simulink model "kapizza_pendulum"  (R2023b)
settings: Solver=VariableStepAuto  StartTime=0.0  StopTime=10  MaxStep=0.01  RelTol=1e-3
values from neighbouring files (symbols this model uses):
  Amplitude = 0.1    [kapizza_script.m]
  decrement = 0.3    [kapizza_script.m]
  Frequency = F_0*30    [kapizza_script.m]
  g = 9.8    [kapizza_script.m]
  L = 1    [kapizza_script.m]
  m = 1    [kapizza_script.m]
  start_angle = 120    [kapizza_script.m]
undefined symbols (not defined in the file or in its folder): I
libraries: simulink_extras x2
settings Model: Creator=user  LastModifiedBy=user
settings DataIOCC: ReturnWorkspaceOutputs=off

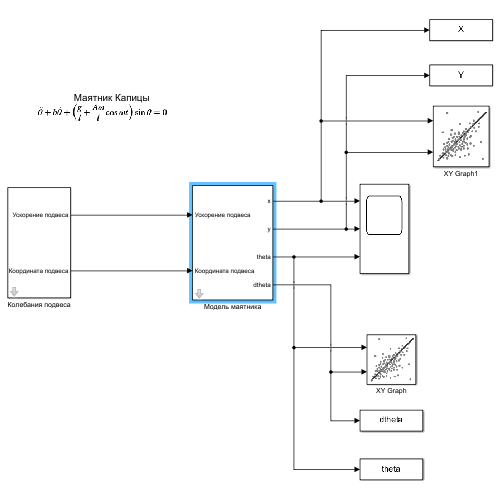
[thumbnail: Simulink's stored preview of the top-level diagram]
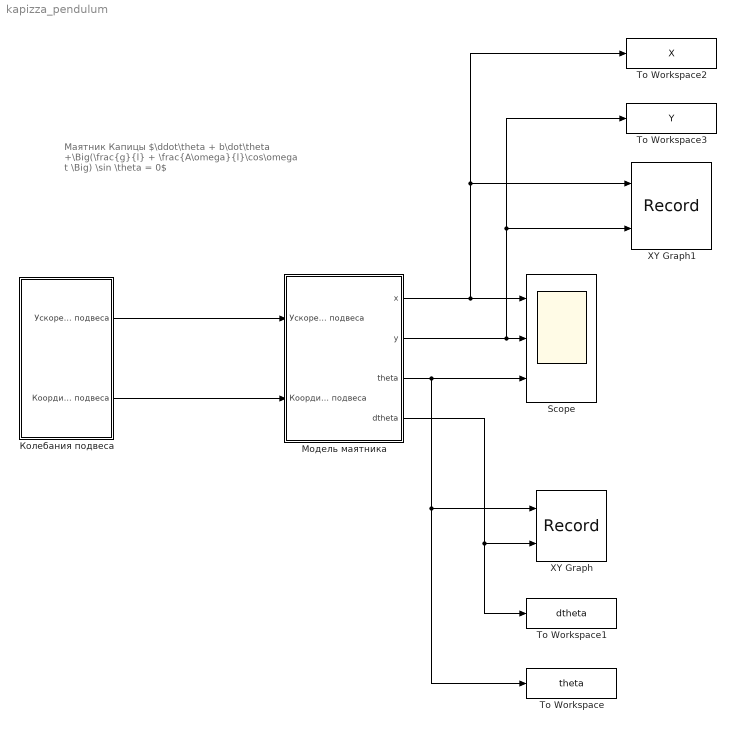
== system kapizza_pendulum ==
  note: Маятник Капицы
      | $\ddot\theta + b\dot\theta +\Big(\frac{g}{l} + \frac{A\omega}{l}\cos\omega t \Big) \sin \theta = 0$
  Scope : Scope  NumInputPorts=3
  To Workspace : ToWorkspace  VariableName=theta  SampleTime=-1
      settings: Save2DSignal=2-D array (concatenate along first dimension)
  To Workspace1 : ToWorkspace  VariableName=dtheta  SampleTime=-1
      settings: Save2DSignal=2-D array (concatenate along first dimension)
  To Workspace2 : ToWorkspace  VariableName=X  SampleTime=-1
      settings: Save2DSignal=2-D array (concatenate along first dimension)
  To Workspace3 : ToWorkspace  VariableName=Y  SampleTime=-1
      settings: Save2DSignal=2-D array (concatenate along first dimension)
  XY Graph : Record  FileSettingsInternal="{\"entries\":[{\"content\":{\"excelSettings\":{\"content\":{},\"type\":\"Streamout.ExcelSettings\"}},\"type\":\"Streamout.FileSettingStorage\",\"uuid\":\"\"}],\"packageUris\":[\"http:\\/\\/schema.mathworks.com\\/mf0\\/streamout_blocks\\/R2020a\"],\"version\":\"1.0\"}"  Layout=[1 1]  SignalsInternal="{\"entries\":[{\"content\":{\"signals\":[{\"content\":{\"blockPath\":[],\"dimensions\":[1],\"domain\":\"\",\"lineColor\":\"#a2142f\",\"plots\":[1],\"port\":1,\"sid\":[\"\"],\"signalID\":1926,\"signalName\":\"Модель маятника:3\"},\"type\":\"RecordBlkView.Signal\",\"uuid\":\"\"},{\"content\":{\"blockPath\":[],\"dimensions\":[1],\"domain\":\"\",\"lineColor\":\"#139fff\",\"plots\":[1],\"port\":2,\"sid\":[\"\"],\"signalID\":1930,\"signalName\":\"Модель маятника:4\"},\"type\":\"RecordBlkView.Signal\",\"uuid\":\"\"}]},\"type\":\"RecordBlkView.InputSignals\",\"uuid\":\"\"}],\"packageUris\":[\"http:\\/\\/schema.mathworks.com\\/mf0\\/streamout_blocks\\/R2020a\"],\"version\":\"1.0\"}"  VisualizationBindings="{\"xyplotplugin\":{\"info\":[{\"series\":[{\"bindingParametersList\":[{\"parameter\":\"X-Axis\",\"signalID\":1926,\"signalName\":\"Модель маятника:3\"},{\"parameter\":\"Y-Axis\",\"signalID\":1930,\"signalName\":\"Модель маятника:4\"}],\"seriesID\":16568}],\"subplotID\":1}]}}"  CompatibilityTag=XY
  XY Graph1 : Record  FileSettingsInternal="{\"entries\":[{\"content\":{\"excelSettings\":{\"content\":{},\"type\":\"Streamout.ExcelSettings\"}},\"type\":\"Streamout.FileSettingStorage\",\"uuid\":\"\"}],\"packageUris\":[\"http:\\/\\/schema.mathworks.com\\/mf0\\/streamout_blocks\\/R2020a\"],\"version\":\"1.0\"}"  Layout=[1 1]  SignalsInternal="{\"entries\":[{\"content\":{\"signals\":[{\"content\":{\"blockPath\":[],\"dimensions\":[1],\"domain\":\"\",\"lineColor\":\"#a2142f\",\"plots\":[1],\"port\":1,\"sid\":[\"\"],\"signalID\":1934,\"signalName\":\"Модель маятника:1\"},\"type\":\"RecordBlkView.Signal\",\"uuid\":\"\"},{\"content\":{\"blockPath\":[],\"dimensions\":[1],\"domain\":\"\",\"lineColor\":\"#139fff\",\"plots\":[1],\"port\":2,\"sid\":[\"\"],\"signalID\":1938,\"signalName\":\"Модель маятника:2\"},\"type\":\"RecordBlkView.Signal\",\"uuid\":\"\"}]},\"type\":\"RecordBlkView.InputSignals\",\"uuid\":\"\"}],\"packageUris\":[\"http:\\/\\/schema.mathworks.com\\/mf0\\/streamout_blocks\\/R2020a\"],\"version\":\"1.0\"}"  VisualizationBindings="{\"xyplotplugin\":{\"info\":[{\"series\":[{\"bindingParametersList\":[{\"parameter\":\"X-Axis\",\"signalID\":1934,\"signalName\":\"Модель маятника:1\"},{\"parameter\":\"Y-Axis\",\"signalID\":1938,\"signalName\":\"Модель маятника:2\"}],\"seriesID\":20568}],\"subplotID\":1}]}}"  CompatibilityTag=XY
  Колебания подвеса : Subsystem  mask{A=Amplitude, f=Frequency}
      mask prompts: A "Амплитуда (м)"; f "Частота (Гц)"
  Модель маятника : Subsystem  mask{m=m, g=g, L=L, start_theta=start_angle, b=decrement}
      mask prompts: m "Масса"; g "Ускорение св. падения"; L "Длина подвеса"; start_theta "Стартовый угол"; b "Коэффициент диссипации"
  wires:
  Модель маятника/3(theta) -> To Workspace/1, XY Graph/1, Scope/3
  Модель маятника/2(y) -> XY Graph1/2, To Workspace3/1, Scope/2
  Модель маятника/1(x) -> XY Graph1/1, To Workspace2/1, Scope/1
  Колебания подвеса/1(Ускорение подвеса) -> Модель маятника/1(Ускорение подвеса)
  Колебания подвеса/2(Координата подвеса) -> Модель маятника/2(Координата подвеса)
  Модель маятника/4(dtheta) -> To Workspace1/1, XY Graph/2

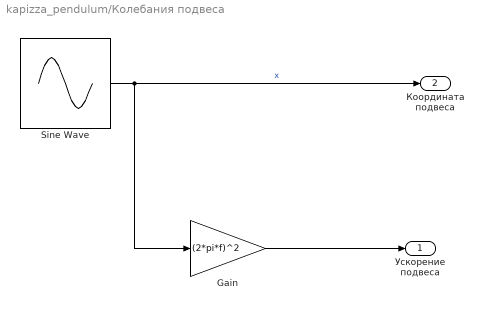
== system kapizza_pendulum/Колебания подвеса ==
  Gain : Gain  Gain=(2*pi*f)^2
  Sine Wave : Sin  Amplitude=A  Frequency=2*pi*f  Phase=pi/2  SampleTime=0
  Ускорение подвеса : Outport
  Координата подвеса : Outport  Port=2
  wires:
  Sine Wave/1 -> Gain/1, Координата подвеса/1  "x"
  Gain/1 -> Ускорение подвеса/1

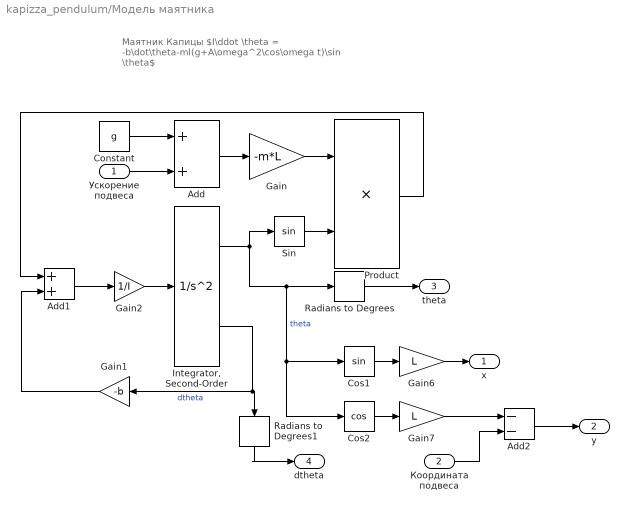
== system kapizza_pendulum/Модель маятника ==
  note: Маятник Капицы
      | $I\ddot \theta = -b\dot\theta-ml(g+A\omega^2\cos\omega t)\sin \theta$
  Ускорение подвеса : Inport
  Координата подвеса : Inport  Port=2
  Add : Sum
  Add1 : Sum
  Add2 : Sum  Inputs=--
  Constant : Constant  Value=g
  Cos1 : Trigonometry
  Cos2 : Trigonometry  Operator=cos
  Gain : Gain  Gain=-m*L
  Gain1 : Gain  Gain=-b
  Gain2 : Gain  Gain=1/I
  Gain6 : Gain  Gain=L
  Gain7 : Gain  Gain=L
  "Integrator, Second-Order" : SecondOrderIntegrator  ICX=deg2rad(start_theta)
  Product : Product
  Radians to Degrees : simulink_extras/Transformations/Radians to Degrees
  Radians to Degrees1 : simulink_extras/Transformations/Radians to Degrees
  Sin : Trigonometry
  x : Outport
  y : Outport  Port=2
  theta : Outport  Port=3
  dtheta : Outport  Port=4
  wires:
  Cos1/1 -> Gain6/1
  Gain6/1 -> x/1
  Cos2/1 -> Gain7/1
  Constant/1 -> Add/1
  Ускорение подвеса/1 -> Add/2
  Add/1 -> Gain/1
  "Integrator, Second-Order"/1 -> Radians to Degrees/1, Cos1/1, Cos2/1, Sin/1  "theta"
  Gain/1 -> Product/1
  Sin/1 -> Product/2
  "Integrator, Second-Order"/2 -> Gain1/1, Radians to Degrees1/1  "dtheta"
  Add1/1 -> Gain2/1
  Gain1/1 -> Add1/2
  Product/1 -> Add1/1
  Gain2/1 -> "Integrator, Second-Order"/1
  Add2/1 -> y/1
  Координата подвеса/1 -> Add2/2
  Gain7/1 -> Add2/1
  Radians to Degrees/1 -> theta/1
  Radians to Degrees1/1 -> dtheta/1
